simulink model "MORSECODEE"  (R2026b)
settings: Solver=FixedStepDiscrete  StopTime=10  FixedStep=0.001
settings Model: Creator=Parth  LastModifiedBy=Parth

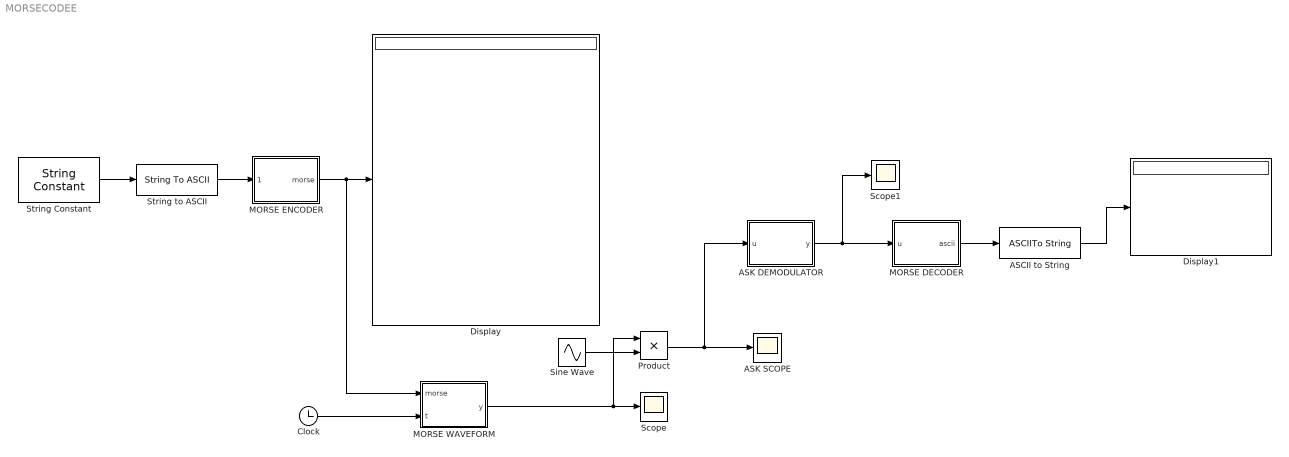
== system MORSECODEE ==
  ASCII to String : ASCIIToString
  ASK DEMODULATOR : MATLAB Function  TreatAsAtomicUnit=on
  ASK SCOPE : Scope
      settings: ActiveDisplayYMinimum=-4.6126936667757743  ActiveDisplayYMaximum=6.47508903866349
  Clock : Clock
  Display : Display
  Display1 : Display
  MORSE DECODER : MATLAB Function  TreatAsAtomicUnit=on
  MORSE ENCODER : MATLAB Function  TreatAsAtomicUnit=on
  MORSE WAVEFORM : MATLAB Function  TreatAsAtomicUnit=on
  Product : Product
  Scope : Scope
      settings: ActiveDisplayYMinimum=-0.12499999999999997  ActiveDisplayYMaximum=1.125
  Scope1 : Scope
      settings: ActiveDisplayYMinimum=-0.12499999999999997  ActiveDisplayYMaximum=1.125  DataLoggingVariableName=ScopeData2
  Sine Wave : Sin  Frequency=628.3185  SampleTime=0.001
  String Constant : StringConstant  String="\"SOS\""
  String to ASCII : StringToASCII
  wires:
  String to ASCII/1 -> MORSE ENCODER/1(message)
  String Constant/1 -> String to ASCII/1
  Clock/1 -> MORSE WAVEFORM/2(t)
  MORSE ENCODER/1(morse) -> MORSE WAVEFORM/1(morse), Display/1
  Sine Wave/1 -> Product/2
  MORSE WAVEFORM/1(y) -> Product/1, Scope/1
  Product/1 -> ASK DEMODULATOR/1(u), ASK SCOPE/1
  ASK DEMODULATOR/1(y) -> MORSE DECODER/1(u), Scope1/1
  MORSE DECODER/1(ascii) -> ASCII to String/1
  ASCII to String/1 -> Display1/1

== matlab function MORSECODEE/MORSE ENCODER ==
  data: message input; morse output
function morse = MorseEncoder(message)

% Output:
% 1 = dot
% 2 = dash
% 0 = gap between elements
% 3 = gap between letters
% 4 = gap between words

% Fixed-size output
morse = zeros(1,100);

p = 1;

for i = 1:length(message)

    ch = message(i);

    % Space = word gap
    if ch == 32

        morse(p) = 4;
        p = p + 1;

    else

        code = getCode(ch);

        for j = 1:length(code)

            if code(j) == 46
                morse(p) = 1;
            elseif code(j) == 45
                morse(p) = 2;
            end

            p = p + 1;

            % Gap between dots/dashes
            if j < length(code)
                morse(p) = 0;
                p = p + 1;
            end

        end

        % Gap between letters
        if i < length(message)
            if message(i+1) ~= 32
                morse(p) = 3;
                p = p + 1;
            end
        end

    end

end


function code = getCode(ch)

switch ch

    case 65, code = '.-';       % A
    case 66, code = '-...';     % B
    case 67, code = '-.-.';     % C
    case 68, code = '-..';      % D
    case 69, code = '.';        % E
    case 70, code = '..-.';     % F
    case 71, code = '--.';      % G
    case 72, code = '....';     % H
    case 73, code = '..';       % I
    case 74, code = '.---';     % J
    case 75, code = '-.-';      % K
    case 76, code = '.-..';     % L
    case 77, code = '--';       % M
    case 78, code = '-.';       % N
    case 79, code = '---';      % O
    case 80, code = '.--.';     % P
    case 81, code = '--.-';     % Q
    case 82, code = '.-.';      % R
    case 83, code = '...';      % S
    case 84, code = '-';        % T
    case 85, code = '..-';      % U
    case 86, code = '...-';     % V
    case 87, code = '.--';      % W
    case 88, code = '-..-';     % X
    case 89, code = '-.--';     % Y
    case 90, code = '--..';     % Z

    case 48, code = '-----';    % 0
    case 49, code = '.----';    % 1
    case 50, code = '..---';    % 2
    case 51, code = '...--';    % 3
    case 52, code = '....-';    % 4
    case 53, code = '.....';    % 5
    case 54, code = '-....';    % 6
    case 55, code = '--...';    % 7
    case 56, code = '---..';    % 8
    case 57, code = '----.';    % 9

    otherwise
        code = '';
end

== matlab function MORSECODEE/ASK DEMODULATOR ==
  data: u input; y output
function y = ASK_Demodulator(u)

persistent buffer index state

if isempty(index)
    buffer = zeros(10,1);
    index = 1;
    state = 0;
end

buffer(index) = abs(u);

if index == 10
    if mean(buffer) > 0.5
        state = 1;
    else
        state = 0;
    end
    index = 1;
else
    index = index + 1;
end

y = state;

end

== matlab function MORSECODEE/MORSE DECODER ==
  data: u input; ascii output
function ascii = MorseDecoder(u)

persistent onTime gapTime symbol result count

if isempty(count)
    onTime = 0;
    gapTime = 0;
    symbol = '';
    result = zeros(1,100,'uint8');
    count = 0;
end

Ts = 0.001;

if u > 0.5
    onTime = onTime + Ts;
    gapTime = 0;

else
    if onTime > 0
        if onTime < 0.2
            symbol = [symbol '.'];
        else
            symbol = [symbol '-'];
        end
        onTime = 0;
    end

    gapTime = gapTime + Ts;

    % Letter gap
    if gapTime >= 0.3 && ~isempty(symbol)

        ch = decodeMorse(symbol);

        if count < 100
            count = count + 1;
            result(count) = uint8(ch);
        end

        symbol = '';
        gapTime = 0;
    end
end

ascii = result;


function ch = decodeMorse(s)

switch s

    case '.-',       ch = 'A';
    case '-...',     ch = 'B';
    case '-.-.',     ch = 'C';
    case '-..',      ch = 'D';
    case '.',        ch = 'E';
    case '..-.',     ch = 'F';
    case '--.',      ch = 'G';
    case '....',     ch = 'H';
    case '..',       ch = 'I';
    case '.---',     ch = 'J';
    case '-.-',      ch = 'K';
    case '.-..',     ch = 'L';
    case '--',       ch = 'M';
    case '-.',       ch = 'N';
    case '---',      ch = 'O';
    case '.--.',     ch = 'P';
    case '--.-',     ch = 'Q';
    case '.-.',      ch = 'R';
    case '...',      ch = 'S';
    case '-',        ch = 'T';
    case '..-',      ch = 'U';
    case '...-',     ch = 'V';
    case '.--',      ch = 'W';
    case '-..-',     ch = 'X';
    case '-.--',     ch = 'Y';
    case '--..',     ch = 'Z';

    case '-----',    ch = '0';
    case '.----',    ch = '1';
    case '..---',    ch = '2';
    case '...--',    ch = '3';
    case '....-',    ch = '4';
    case '.....',    ch = '5';
    case '-....',    ch = '6';
    case '--...',    ch = '7';
    case '---..',    ch = '8';
    case '----.',    ch = '9';

    otherwise
        ch = ' ';

end

== matlab function MORSECODEE/MORSE WAVEFORM ==
  data: morse input; y output; t input
function y = MorseWaveform(morse,t)

unit = 0.1;
y = 0;
currentTime = 0;

for i = 1:length(morse)

    code = morse(i);

    if code == 1
        duration = unit;
        signal = 1;

    elseif code == 2
        duration = 3 * unit;
        signal = 1;

    elseif code == 0
        duration = unit;
        signal = 0;

    elseif code == 3
        duration = 3 * unit;
        signal = 0;

    elseif code == 4
        duration = 7 * unit;
        signal = 0;

    else
        duration = 0;
        signal = 0;
    end

    if t >= currentTime && t < currentTime + duration
        y = signal;
        return;
    end

    currentTime = currentTime + duration;

end
